simulink model "gimbal_2axis"  (R2024a)
settings: Solver=FixedStepDiscrete  StartTime=0.0  StopTime=4  FixedStep=0.002  RelTol=1e-3
model workspace (MAT data in the model file):
  P.Ts = 0.002
  P.Kt = 0.741
  P.Imax = 3
  P.Jyaw = 0.015
  P.Jpitch = 0.008
  P.Byaw = 0.035
  P.Bpitch = 0.025
  P.pitchGravity = 0.08
  P.yawLadrc = [4 500 8 32 1]
  P.pitchLadrc = [2.5 120 1.5 3 0.03]
  P.pitchEnabled = 1
values from neighbouring files (symbols this model uses):
  P = getVariable(get_param(model, 'ModelWorkspace'), 'P')    [run_gimbal_sim.m]
settings Model: Creator=www  LastModifiedBy=www

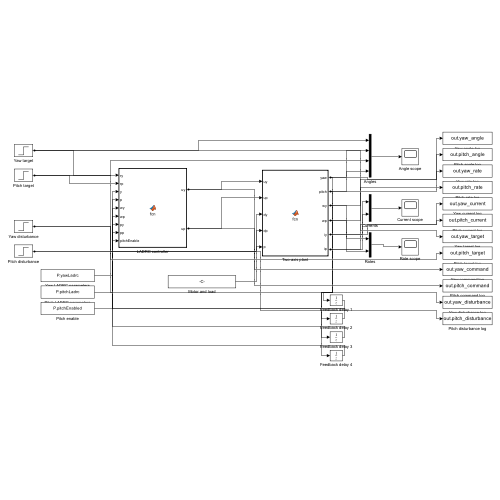
[thumbnail: Simulink's stored preview of the top-level diagram]
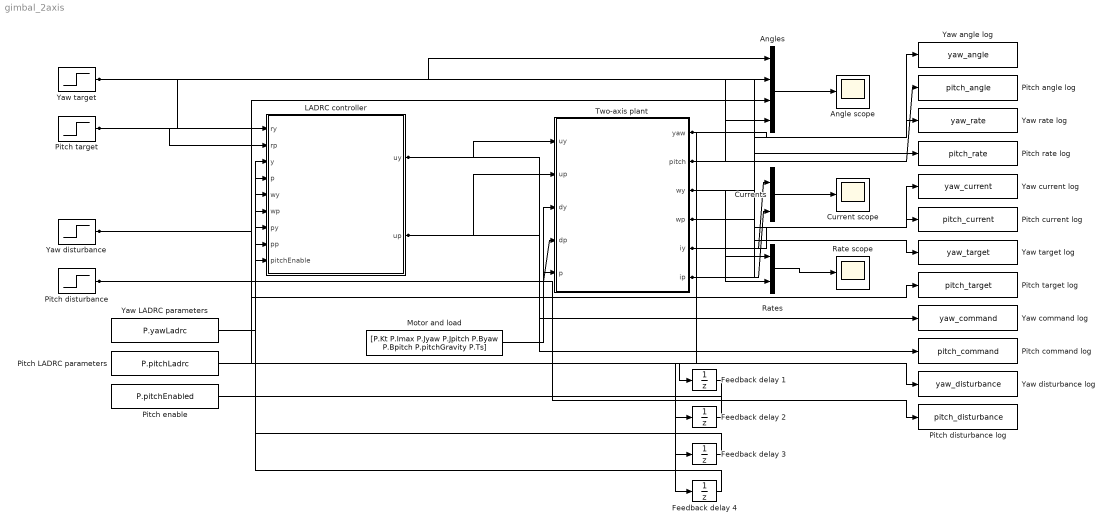
== system gimbal_2axis ==
  Angle scope : Scope
  Angles : Mux
  Current scope : Scope
  Currents : Mux  Inputs=2
  Feedback delay {1..4} (4 alike) : UnitDelay  SampleTime=P.Ts  HasFrameUpgradeWarning=on
  LADRC controller : MATLAB Function  TreatAsAtomicUnit=on
  Motor and load : Constant  Value=[P.Kt P.Imax P.Jyaw P.Jpitch P.Byaw P.Bpitch P.pitchGravity P.Ts]
  Pitch LADRC parameters : Constant  Value=P.pitchLadrc
  Pitch angle log : ToWorkspace  VariableName=pitch_angle  SaveFormat=Timeseries  SampleTime=-1
  Pitch command log : ToWorkspace  VariableName=pitch_command  SaveFormat=Timeseries  SampleTime=-1
  Pitch current log : ToWorkspace  VariableName=pitch_current  SaveFormat=Timeseries  SampleTime=-1
  Pitch disturbance : Step  Time=2.7  After=0.04  SampleTime=P.Ts
  Pitch disturbance log : ToWorkspace  VariableName=pitch_disturbance  SaveFormat=Timeseries  SampleTime=-1
  Pitch enable : Constant  Value=P.pitchEnabled
  Pitch rate log : ToWorkspace  VariableName=pitch_rate  SaveFormat=Timeseries  SampleTime=-1
  Pitch target : Step  After=0.25  SampleTime=P.Ts
  Pitch target log : ToWorkspace  VariableName=pitch_target  SaveFormat=Timeseries  SampleTime=-1
  Rate scope : Scope
  Rates : Mux  Inputs=2
  Two-axis plant : MATLAB Function  TreatAsAtomicUnit=on
  Yaw LADRC parameters : Constant  Value=P.yawLadrc
  Yaw angle log : ToWorkspace  VariableName=yaw_angle  SaveFormat=Timeseries  SampleTime=-1
  Yaw command log : ToWorkspace  VariableName=yaw_command  SaveFormat=Timeseries  SampleTime=-1
  Yaw current log : ToWorkspace  VariableName=yaw_current  SaveFormat=Timeseries  SampleTime=-1
  Yaw disturbance : Step  Time=2.3  After=0.06  SampleTime=P.Ts
  Yaw disturbance log : ToWorkspace  VariableName=yaw_disturbance  SaveFormat=Timeseries  SampleTime=-1
  Yaw rate log : ToWorkspace  VariableName=yaw_rate  SaveFormat=Timeseries  SampleTime=-1
  Yaw target : Step  Time=0.5  After=0.6  SampleTime=P.Ts
  Yaw target log : ToWorkspace  VariableName=yaw_target  SaveFormat=Timeseries  SampleTime=-1
  wires:
  Yaw target/1 -> LADRC controller/1(ry), Angles/1, Yaw target log/1
  Pitch target/1 -> LADRC controller/2(rp), Angles/3, Pitch target log/1
  Two-axis plant/1(yaw) -> Feedback delay 1/1, Angles/2, Yaw angle log/1
  Feedback delay 1/1 -> LADRC controller/3(y)
  Two-axis plant/2(pitch) -> Feedback delay 2/1, Angles/4, Pitch angle log/1
  Feedback delay 2/1 -> LADRC controller/4(p)
  Two-axis plant/3(wy) -> Feedback delay 3/1, Rates/1, Yaw rate log/1
  Feedback delay 3/1 -> LADRC controller/5(wy)
  Two-axis plant/4(wp) -> Feedback delay 4/1, Rates/2, Pitch rate log/1
  Feedback delay 4/1 -> LADRC controller/6(wp)
  Yaw LADRC parameters/1 -> LADRC controller/7(py)
  Pitch LADRC parameters/1 -> LADRC controller/8(pp)
  Pitch enable/1 -> LADRC controller/9(pitchEnable)
  LADRC controller/1(uy) -> Two-axis plant/1(uy), Yaw command log/1
  LADRC controller/2(up) -> Two-axis plant/2(up), Pitch command log/1
  Yaw disturbance/1 -> Two-axis plant/3(dy), Yaw disturbance log/1
  Pitch disturbance/1 -> Two-axis plant/4(dp), Pitch disturbance log/1
  Motor and load/1 -> Two-axis plant/5(p)
  Angles/1 -> Angle scope/1
  Two-axis plant/5(iy) -> Currents/1, Yaw current log/1
  Two-axis plant/6(ip) -> Currents/2, Pitch current log/1
  Currents/1 -> Current scope/1
  Rates/1 -> Rate scope/1

== matlab function gimbal_2axis/Two-axis plant ==
  data: uy input; yaw output; up input; dy input; dp input; p input; pitch output; wy output; wp output; iy output; ip output
function [yaw,pitch,wy,wp,iy,ip] = fcn(uy,up,dy,dp,p)
%#codegen
% Fixed-step surrogate: no measured assembly inertia or inner-loop model.
persistent x
if isempty(x), x=zeros(1,4); end
yaw=x(1); pitch=x(2); wy=x(3); wp=x(4);
iy=min(max(uy,-1),1)*p(2);
ip=min(max(up,-1),1)*p(2);
tauY=p(1)*iy+dy;
tauP=p(1)*ip+dp-p(7)*sin(pitch);
ay=(tauY-p(5)*wy)/p(3);
ap=(tauP-p(6)*wp)/p(4);
x(3)=wy+p(8)*ay; x(4)=wp+p(8)*ap;
x(1)=yaw+p(8)*x(3); x(2)=pitch+p(8)*x(4);
end

== matlab function gimbal_2axis/LADRC controller ==
  data: ry input; uy output; rp input; y input; p input; wy input; wp input; py input; pp input; pitchEnable input; up output
function [uy,up] = fcn(ry,rp,y,p,wy,wp,py,pp,pitchEnable)
%#codegen
% The active firmware uses yaw LADRC; Pitch is an optional experiment.
persistent sy sp wasOn
if isempty(wasOn)
    sy = zeros(1,11); sp = zeros(1,11); wasOn = false;
end
if ~wasOn
    sy = [y wy y wy 0 0 0 0 0 0 0];
    sp = [p wp p wp 0 0 0 0 0 0 0];
    wasOn = true;
end
% Pitch software limit and the Euler singularity protection.
rp = min(max(rp,-1.22173048),1.22173048);
if abs(p)>1.22173048
    uy=0; up=0; wasOn=false; return;
end
[uy,sy] = axisStep(ry,y,sy,py,0.002);
if pitchEnable~=0
    [up,sp] = axisStep(rp,p,sp,pp,0.002);
else
    up = 0;
end
end
function [u,s] = axisStep(ref,fb,s,q,T)
% State: v1 v2 z1 z2 z3 and prior derivatives, prior command.
halfT = 0.5*T;
fbContinuous = s(3)+circleError(fb,s(3));
refContinuous = fbContinuous+circleError(ref,fb);
r=q(1); b0=q(2); wc=q(3); w0=q(4); limit=q(5);
fh = -r*r*(s(1)-refContinuous)-2*r*s(2);
s(2) = s(2)+halfT*(fh+s(7));
s(1) = s(1)+halfT*(s(2)+s(6));
s(7) = fh; s(6) = s(2);
e = s(3)-fbContinuous;
dz3 = -w0*w0*w0*e;
dz2 = s(5)-3*w0*w0*e+b0*s(11);
dz1 = s(4)-3*w0*e;
s(5) = s(5)+halfT*(dz3+s(10));
s(4) = s(4)+halfT*(dz2+s(9));
s(3) = s(3)+halfT*(dz1+s(8));
s(10)=dz3; s(9)=dz2; s(8)=dz1;
u = (wc*wc*(s(1)-s(3))+2*wc*(s(2)-s(4))-s(5))/b0;
if ~isfinite(u) || ~all(isfinite(s))
    s=[fb 0 fb 0 0 0 0 0 0 0 0]; u=0;
end
u = min(max(u,-limit),limit); s(11)=u;
end
function e = circleError(a,b)
e=a-b;
if e>pi, e=e-2*pi; elseif e<-pi, e=e+2*pi; end
end
